simulink model "TP_manual_offline"  (R2024b)
settings: Solver=ode4  StartTime=0.0  StopTime=T_end_tp  FixedStep=Ts_tp  RelTol=1e-3
PostLoadFcn:
  | addpath(fileparts(get_param('TP_manual_offline','FileName')));
InitFcn:
  | TP_manual_init('TP_manual_offline');
StopFcn:
  | TP_manual_stop('TP_manual_offline');
values from neighbouring files (symbols this model uses):
  alloc_prm = [half_beam; l_bow; F_max; F_bow_max]    [TP_manual_setup.m]
  D = G.D(1:G.n, :)    [TP_gcs.m]
  N_btn = 400    [TP_manual_setup.m]
  S = struct('n', 0)    [TP_gcs.m]    (also in TP_manual_check.m = TP_gcs('result'); TP_manual_stop.m = TP_gcs('result'); TP_mission.m = TP_gcs('result'))
  Ts_tp = 0.05    [TP_manual_setup.m]
  usv_p = [m_usv; Izz; Xu; Xuu; Yv; Yvv; Nr; Nrr; half_beam; l_bow]    [TP_manual_setup.m]
  W = 1 - e2*sind(lat0)^2    [TP_gcs.m]    (also in TP_make_video.m = [])
  x0_tp = [0; 0; 0; -32; 0; 0]    [TP_manual_setup.m]
  X_btn = 400    [TP_manual_setup.m]
  Y_btn = 200    [TP_manual_setup.m]
undefined symbols (not defined in the file or in its folder): A, Q
settings Model: Creator=wkyou  LastModifiedBy=wkyou

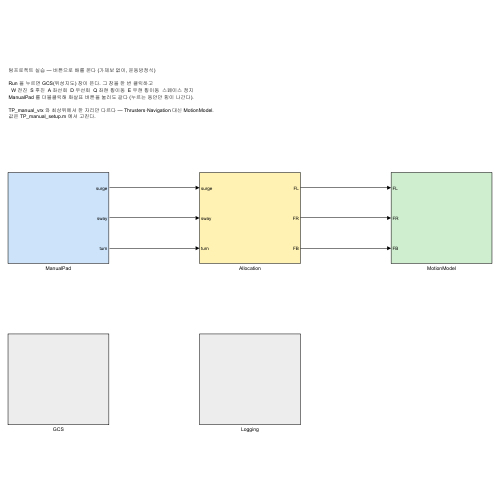
[thumbnail: Simulink's stored preview of the top-level diagram]
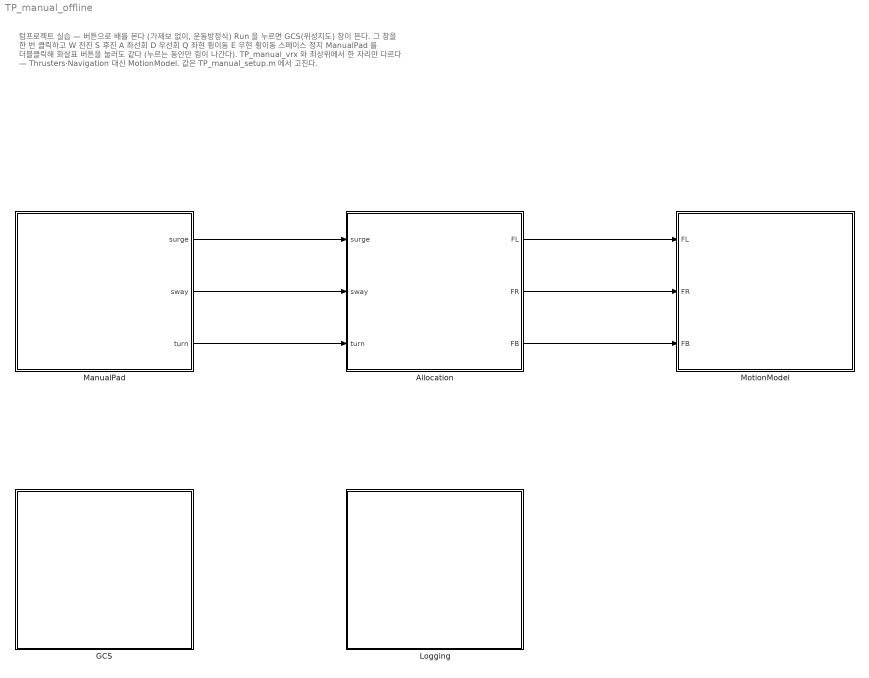
== system TP_manual_offline ==
  note: 텀프로젝트 실습 — 버튼으로 배를 몬다 (가제보 없이, 운동방정식)
      |
      | Run 을 누르면 GCS(위성지도) 창이 뜬다. 그 창을 한 번 클릭하고
      |   W 전진  S 후진  A 좌선회  D 우선회  Q 좌현 횡이동  E 우현 횡이동  스페이스 정지
      | ManualPad 를 더블클릭해 화살표 버튼을 눌러도 같다 (누르는 동안만 힘이 나간다).
      |
      | TP_manual_vrx 와 최상위에서 한 자리만 다르다 — Thrusters·Navigation 대신 MotionModel.
      | 값은 TP_manual_setup.m 에서 고친다.
  Allocation : Subsystem
  GCS : Subsystem
  Logging : Subsystem
  ManualPad : Subsystem
  MotionModel : Subsystem
  wires:
  ManualPad/1(surge) -> Allocation/1(surge)
  Allocation/1(FL) -> MotionModel/1(FL)
  ManualPad/2(sway) -> Allocation/2(sway)
  Allocation/2(FR) -> MotionModel/2(FR)
  ManualPad/3(turn) -> Allocation/3(turn)
  Allocation/3(FB) -> MotionModel/3(FB)

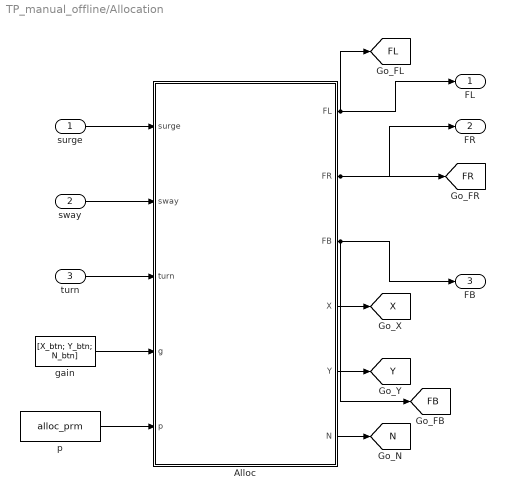
== system TP_manual_offline/Allocation ==
  surge : Inport
  sway : Inport  Port=2
  turn : Inport  Port=3
  Alloc : MATLAB Function  TreatAsAtomicUnit=on
  gain : Constant  Value=[X_btn; Y_btn; N_btn]
  p : Constant  Value=alloc_prm
  FL : Outport
  FR : Outport  Port=2
  FB : Outport  Port=3
  tag scope: FB=global, FL=global, FR=global, N=global, X=global, Y=global
  wires:
  surge/1 -> Alloc/1(surge)
  Alloc/3(FB) -> FB/1, [FB]
  sway/1 -> Alloc/2(sway)
  turn/1 -> Alloc/3(turn)
  Alloc/1(FL) -> FL/1, [FL]
  p/1 -> Alloc/5(p)
  gain/1 -> Alloc/4(g)
  Alloc/2(FR) -> [FR], FR/1
  Alloc/6(N) -> [N]
  Alloc/4(X) -> [X]
  Alloc/5(Y) -> [Y]

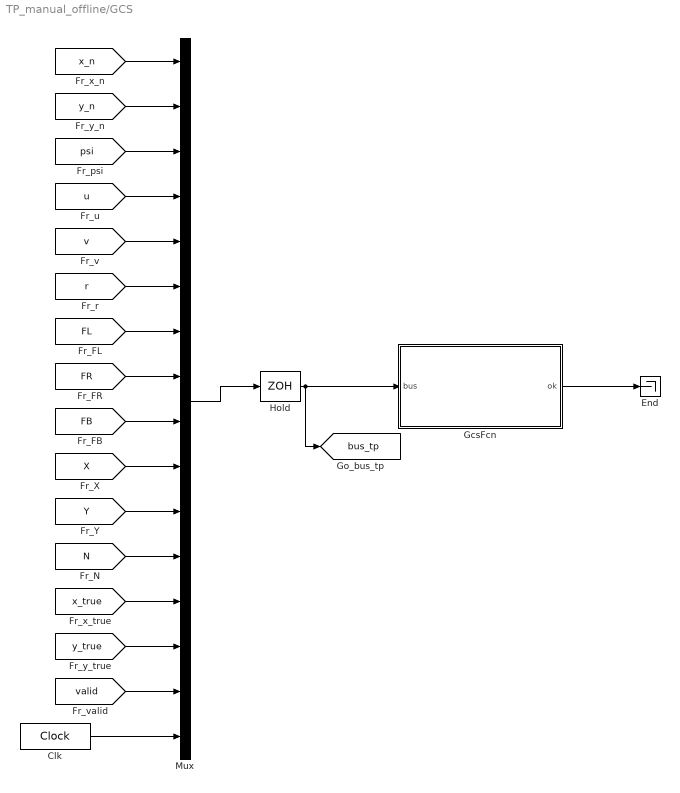
== system TP_manual_offline/GCS ==
  Clk : DigitalClock  SampleTime=Ts_tp
  End : Terminator
  GcsFcn : MATLAB Function  TreatAsAtomicUnit=on
  Hold : ZeroOrderHold  SampleTime=Ts_tp
  Mux : Mux  Inputs=16
  tag scope: bus_tp=global
  wires:
  Clk/1 -> Mux/16
  Mux/1 -> Hold/1
  Hold/1 -> GcsFcn/1(bus), [bus_tp]
  GcsFcn/1(ok) -> End/1
  [FB] -> Mux/9
  [FL] -> Mux/7
  [FR] -> Mux/8
  [N] -> Mux/12
  [X] -> Mux/10
  [Y] -> Mux/11
  [psi] -> Mux/3
  [r] -> Mux/6
  [u] -> Mux/4
  [v] -> Mux/5
  [valid] -> Mux/15
  [x_n] -> Mux/1
  [x_true] -> Mux/13
  [y_n] -> Mux/2
  [y_true] -> Mux/14

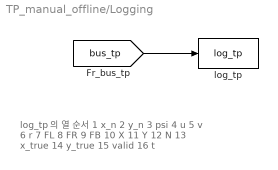
== system TP_manual_offline/Logging ==
  note: log_tp 의 열 순서
      |  1 x_n   2 y_n   3 psi   4 u   5 v   6 r
      |  7 FL    8 FR    9 FB   10 X  11 Y  12 N
      | 13 x_true  14 y_true  15 valid  16 t
  log_tp : ToWorkspace  VariableName=log_tp  SaveFormat=Timeseries  SampleTime=Ts_tp
  wires:
  [bus_tp] -> log_tp/1

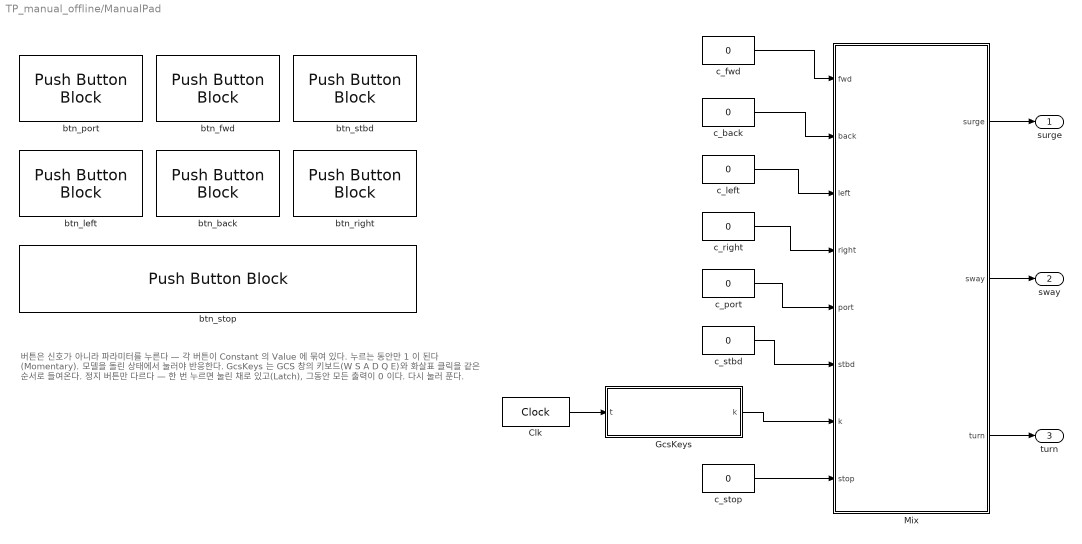
== system TP_manual_offline/ManualPad ==
  note: 버튼은 신호가 아니라 파라미터를 누른다 — 각 버튼이 Constant 의 Value 에 묶여 있다.
      | 누르는 동안만 1 이 된다 (Momentary). 모델을 돌린 상태에서 눌러야 반응한다.
      | GcsKeys 는 GCS 창의 키보드(W S A D Q E)와 화살표 클릭을 같은 순서로 들여온다.
      | 정지 버튼만 다르다 — 한 번 누르면 눌린 채로 있고(Latch), 그동안 모든 출력이 0 이다. 다시 눌러 푼다.
  Clk : DigitalClock  SampleTime=Ts_tp
  GcsKeys : MATLAB Function  TreatAsAtomicUnit=on
  Mix : MATLAB Function  TreatAsAtomicUnit=on
  btn_back : PushButtonBlock  ButtonText=▼ 후진 (S)
  btn_fwd : PushButtonBlock  ButtonText=▲ 전진 (W)
  btn_left : PushButtonBlock  ButtonText=◀ 좌선회 (A)
  btn_port : PushButtonBlock  ButtonText=⇦ 좌현 횡 (Q)
  btn_right : PushButtonBlock  ButtonText=▶ 우선회 (D)
  btn_stbd : PushButtonBlock  ButtonText=⇨ 우현 횡 (E)
  btn_stop : PushButtonBlock  ButtonText="■ 정지 — 모든 출력 0  (다시 누르면 풀림)"  ButtonType=Latch
  c_back : Constant  Value=0
  c_fwd : Constant  Value=0
  c_left : Constant  Value=0
  c_port : Constant  Value=0
  c_right : Constant  Value=0
  c_stbd : Constant  Value=0
  c_stop : Constant  Value=0
  surge : Outport
  sway : Outport  Port=2
  turn : Outport  Port=3
  wires:
  Clk/1 -> GcsKeys/1(t)
  c_right/1 -> Mix/4(right)
  c_fwd/1 -> Mix/1(fwd)
  c_back/1 -> Mix/2(back)
  c_port/1 -> Mix/5(port)
  c_left/1 -> Mix/3(left)
  Mix/1(surge) -> surge/1
  c_stbd/1 -> Mix/6(stbd)
  GcsKeys/1(k) -> Mix/7(k)
  c_stop/1 -> Mix/8(stop)
  Mix/2(sway) -> sway/1
  Mix/3(turn) -> turn/1

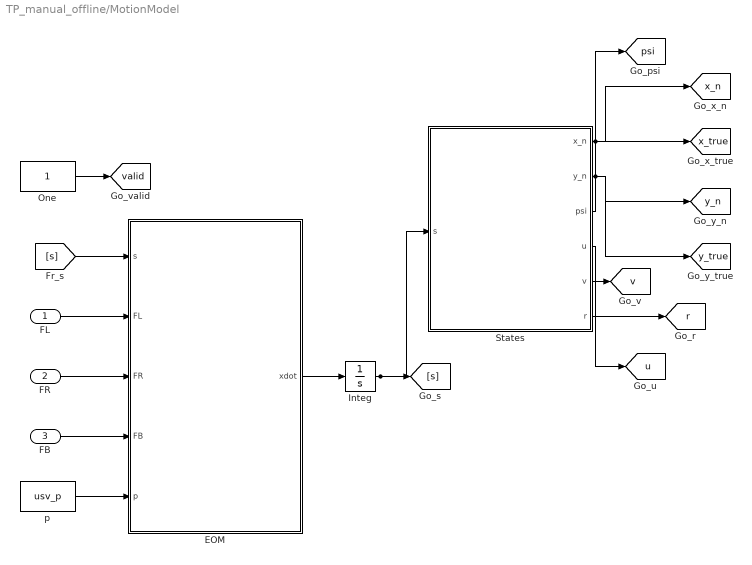
== system TP_manual_offline/MotionModel ==
  FL : Inport
  FR : Inport  Port=2
  FB : Inport  Port=3
  EOM : MATLAB Function  TreatAsAtomicUnit=on
  Integ : Integrator  InitialCondition=x0_tp
  One : Constant
  States : MATLAB Function  TreatAsAtomicUnit=on
  p : Constant  Value=usv_p
  tag scope: psi=global, r=global, u=global, v=global, valid=global, x_n=global, x_true=global, y_n=global, y_true=global
  wires:
  Integ/1 -> States/1(s), [s]
  FL/1 -> EOM/2(FL)
  FR/1 -> EOM/3(FR)
  FB/1 -> EOM/4(FB)
  EOM/1(xdot) -> Integ/1
  p/1 -> EOM/5(p)
  One/1 -> [valid]
  [s] -> EOM/1(s)
  States/2(y_n) -> [y_n], [y_true]
  States/1(x_n) -> [x_n], [x_true]
  States/3(psi) -> [psi]
  States/6(r) -> [r]
  States/4(u) -> [u]
  States/5(v) -> [v]

== matlab function TP_manual_offline/ManualPad/Mix ==
  data: fwd input; surge output; back input; left input; right input; port input; stbd input; k input; stop input; sway output; turn output
function [surge, sway, turn] = Mix(fwd, back, left, right, port, stbd, k, stop)
%#codegen
% 버튼 여섯(이 상자의 Push Button)과 GCS 창의 입력 k 를 합친다.
% 어느 쪽에서 누르든 같다 — 하나라도 눌리면 1.
b = min(1, [fwd; back; left; right; port; stbd] + k);

surge = b(1) - b(2);     % 전진 +1, 후진 -1
sway  = b(6) - b(5);     % 우현 +1, 좌현 -1   (선수추진기가 맡는다)
turn  = b(4) - b(3);     % 우선회 +1 (시계방향), 좌선회 -1

% 정지 버튼이 눌려 있으면 무엇이 눌렸든 0 을 낸다 — 추력 셋이 모두 0 이 된다
if stop > 0.5
    surge = 0;  sway = 0;  turn = 0;
end

== matlab function TP_manual_offline/ManualPad/GcsKeys ==
  data: t input; k output
function k = GcsKeys(t)
%#codegen
% GCS 창에서 눌린 조종 입력을 읽는다 (TP_gcs_keys.m).
%   k = [전진; 후진; 좌선회; 우선회; 좌현 횡이동; 우현 횡이동],  각 0 또는 1
% 그림 창의 값이라 코드 생성 대상이 아니다. extrinsic 으로 부른다.
coder.extrinsic('TP_gcs_keys');
k = zeros(6, 1);
k = TP_gcs_keys(t);

== matlab function TP_manual_offline/Allocation/Alloc ==
  data: surge input; FL output; sway input; turn input; g input; p input; FR output; FB output; X output; Y output; N output
function [FL, FR, FB, X, Y, N] = Alloc(surge, sway, turn, g, p)
%#codegen
% 1) 버튼 값(-1 · 0 · +1)에 힘을 곱해 요구 힘·모멘트를 만든다
%      g = [X_btn; Y_btn; N_btn]   버튼 하나가 요구하는 힘 (TP_manual_setup.m)
X = g(1)*surge;          % 전후력 [N]      앞 +
Y = g(2)*sway;           % 횡력 [N]        우현 +
N = g(3)*turn;           % 요 모멘트 [N m] 시계방향 +

% 2) 추력 배분 — 세 추진기로 나눈다 (6주차 W06 의 배분식 그대로)
%      X = FL + FR
%      Y = FB                           횡력은 선수추진기만 낸다
%      N = (FL - FR)*b + l3*FB
%    p = [b; l3; Fmax; Fbmax]
%      b   좌·우 추진기까지의 반폭 [m],  l3  선수추진기의 앞쪽 거리 [m]
%
%    선수추진기가 횡력을 내면 요 모멘트 l3*FB 가 딸려 온다. 그 몫을 좌·우
%    추진기가 되받아 빼야 선수각이 돌지 않는다 — 아래 N - l3*FB 가 그것이다.
b = p(1);  l3 = p(2);  Fmax = p(3);  Fbmax = p(4);
FB = min(max(Y, -Fbmax), Fbmax);
M  = N - l3*FB;          % 포화된 뒤의 FB 로 센다 — 실제로 딸려 온 만큼만 되받는다
FL = X/2 + M/(2*b);
FR = X/2 - M/(2*b);
FL = min(max(FL, -Fmax), Fmax);
FR = min(max(FR, -Fmax), Fmax);

== matlab function TP_manual_offline/MotionModel/EOM ==
  data: s input; xdot output; FL input; FR input; FB input; p input
function xdot = EOM(s, FL, FR, FB, p)
%#codegen
% 3 자유도 운동방정식 (NED).  s = [u v r x_n y_n psi]'
%   계수는 VRX 설정파일에서 읽은 값이다 (6주차 W06_setup.m 과 같다)
%   p = [m Izz Xu Xuu Yv Yvv Nr Nrr b l3]'
u = s(1);  v = s(2);  r = s(3);  psi = s(6);
m_s = p(1);  Izz = p(2);  Xu = p(3);  Xuu = p(4);  Yv = p(5);  Yvv = p(6);
Nr = p(7);  Nrr = p(8);  b_h = p(9);  l3 = p(10);

% 추진기 셋이 내는 힘과 모멘트
X = FL + FR;
Y = FB;
N = (FL - FR)*b_h + l3*FB;

% 저항 — 선형 + 제곱
Dx = (Xu + Xuu*abs(u))*u;
Dy = (Yv + Yvv*abs(v))*v;
Dn = (Nr + Nrr*abs(r))*r;

du = (X - Dx)/m_s + v*r;
dv = (Y - Dy)/m_s - u*r;
dr = (N - Dn)/Izz;

xdot = [du; dv; dr; ...
        u*cos(psi) - v*sin(psi); ...
        u*sin(psi) + v*cos(psi); ...
        r];

== matlab function TP_manual_offline/MotionModel/States ==
  data: s input; x_n output; y_n output; psi output; u output; v output; r output
function [x_n, y_n, psi, u, v, r] = States(s)
%#codegen
% 상태 벡터 s = [u v r x_n y_n psi] 를 이름 있는 신호로 꺼낸다.
% psi 는 적분값이라 한 바퀴 돌면 2*pi 를 넘는다. -pi..pi 로 접는다.
u = s(1);  v = s(2);  r = s(3);
x_n = s(4);  y_n = s(5);
psi = atan2(sin(s(6)), cos(s(6)));

== matlab function TP_manual_offline/GCS/GcsFcn ==
  data: bus input; ok output
function ok = GcsFcn(bus)
%#codegen
% GCS 창(위성지도·그래프·조종 버튼)을 부른다 — TP_gcs.m
%   bus = [x_n y_n psi u v r FL FR FB X Y N x_true y_true valid  t]
% 그림은 코드 생성 대상이 아니므로 extrinsic 으로 부른다.
coder.extrinsic('TP_gcs');
ok = 1;
TP_gcs(bus(1:15), bus(16));
